simulink model "frequency_FPID_offline"  (R2025b)
settings: Solver=ode45  StartTime=0.0  StopTime=40  RelTol=1e-3
undefined symbols (not defined in the file): B1, B2, DBH1, DBH2, dbpu, GRCT1, GRCU1, KBESS, KD1, Kd1_RL, Kd2_RL, KDeng, Ke, Kev, KH1, Ki1_RL, Ki2_RL, KP, KP1, Kp1_RL, KP2, Kp2_RL, Kpc, KPV1, KPV2, Kr1, KT1, KW, Kw1, Kw2, KX1_RL, KX2_RL, KY1_RL, KY2_RL, N1, N2, Nev, PAGmax, PAGmin, R1, R2, Rev, T12, TBESS, Td0, Td1, Td2, Td3, Tev, TG1, Th1, Th2, TP1, TP2, Tpt1, Tpt2, TPV1, TPV2, Tr1, Trh1 ... (+9)
libraries: fuzblock x2, slpidlib x2, simulink x2

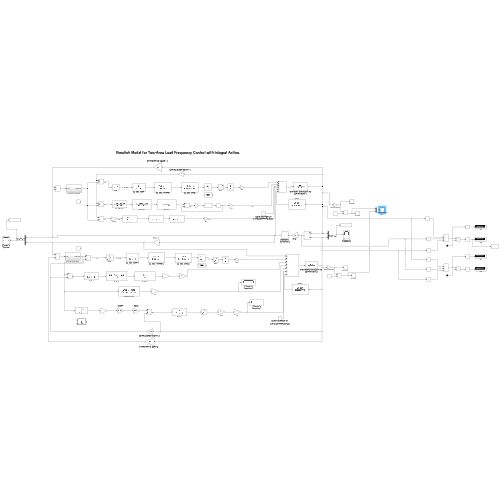
[thumbnail: Simulink's stored preview of the top-level diagram]
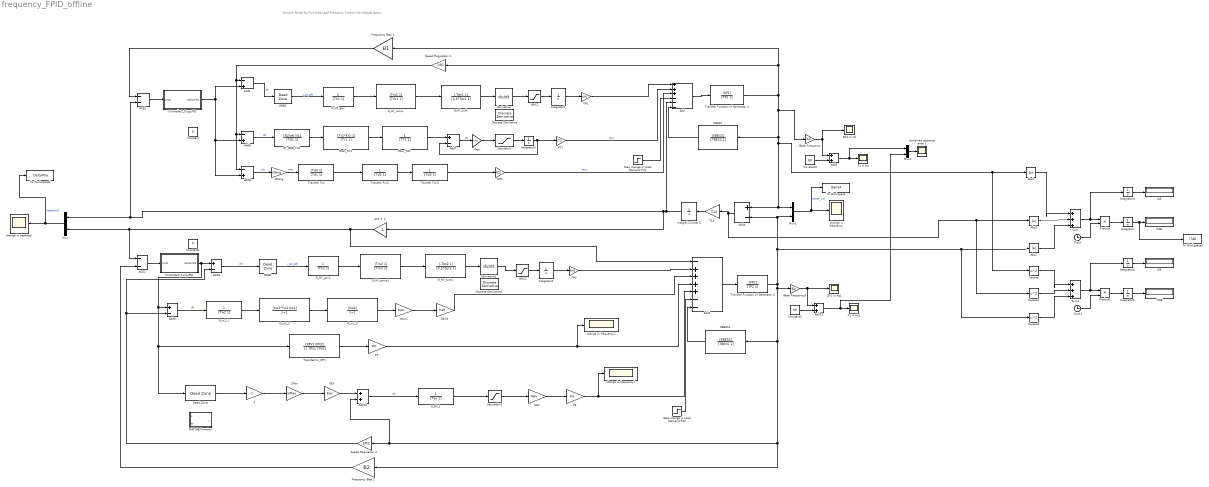
== system frequency_FPID_offline ==
  note: Simulink Model for Two-Area Load Frequency Control with Integral Action.
  " change in frequency" : Scope
      settings: ActiveDisplayYMinimum=-0.0040302316669391719  ActiveDisplayYMaximum=0.00095804845606976461
  " change in frequency1" : Scope
      settings: ActiveDisplayYMinimum=-0.00030105594584369807  ActiveDisplayYMaximum=4.6057283791285268E-5  DataLoggingVariableName=ScopeData3
  " change in frequency2" : Scope
      settings: ActiveDisplayYMinimum=-0.0033871282854349067  ActiveDisplayYMaximum=0.00055417492830862479  DataLoggingVariableName=ScopeData4
  " change in tiepower" : Scope
      settings: ActiveDisplayYMinimum=-0.0024845401904889861  ActiveDisplayYMaximum=0.0033711842064116687
  -1 : Gain  Gain=-1
  1/Rev : Gain  Gain=1/Rev
  A12 = 1 : Gain  Gain=-1
  ACE1 : Sum  Inputs=--
  ACE2 : Sum  Inputs=--
  Abs1 : Abs  SaturateOnIntegerOverflow=off
  Abs2 : Abs  SaturateOnIntegerOverflow=off
  Abs3 : Abs  SaturateOnIntegerOverflow=off
  Add : Sum  Inputs=+++---
  Add1 : Sum  Inputs=-+
  Add10 : Sum
  Add12 : Sum
  Add2 : Sum  Inputs=-++++--
  Add{3..4,7,9} (4 alike) : Sum  Inputs=+-
  Add5 : Sum
  Add6 : Sum  Inputs=-+
  Add8 : Sum  Inputs=-+
  Base Frequency : Gain  Gain=60
  Base Frequency2 : Gain  Gain=60
  Clock : Clock
  Clock1 : Clock
  Constant : Constant  Value=0
  Constant1 : Constant  Value=0
  Constant2 : Constant  Value=60
  Constant3 : Constant  Value=60
  Controller1_FuzzyPID : Subsystem
  Controller2_FuzzyPID : Subsystem
  DF1 in Hz : Scope
      settings: ActiveDisplayYMinimum=-0.70637481280735892  ActiveDisplayYMaximum=0.1303080522857864  DataLoggingVariableName=ScopeData5
  DF1 in Hz1 : Scope
      settings: ActiveDisplayYMinimum=-0.88482  ActiveDisplayYMaximum=0.09831  DataLoggingVariableName=ScopeData2
  Dead Zone : DeadZone  LowerValue=-dbpu  UpperValue=+dbpu
  Derivative : Derivative
  Derivative1 : Derivative
  Discrete Derivative : simulink/Discrete/Discrete Derivative  gainval=1.0  ICPrevScaledInput=0.0  OutMin=[]  OutMax=[]  OutDataType=fixdt(1, 16)  OutScaling=2^-10  DoSatur=off
  Discrete Derivative1 : simulink/Discrete/Discrete Derivative  gainval=1.0  ICPrevScaledInput=0.0  OutMin=[]  OutMax=[]  OutDataType=fixdt(1, 16)  OutScaling=2^-10  DoSatur=off
  F1 in Hz : Scope
      settings: ActiveDisplayYMinimum=59.317272894162173  ActiveDisplayYMaximum=60.108382672060813  DataLoggingVariableName=ScopeData7
  F1 in Hz1 : Scope
      settings: ActiveDisplayYMinimum=59.53516  ActiveDisplayYMaximum=60.11035  DataLoggingVariableName=ScopeData9
  Frequency Bias 1 : Gain  Gain=B1
  Frequency Bias 2 : Gain  Gain=B2
  GBESS : TransferFcn  Numerator=[KBESS]  Denominator=[TBESS 1]
  GBESS1 : TransferFcn  Numerator=[KBESS]  Denominator=[TBESS 1]
  GDB1 : DeadZone  LowerValue=-DBH1  UpperValue=+DBH1  ZeroCross=off
  GDB2 : DeadZone  LowerValue=-DBH2  UpperValue=+DBH2  ZeroCross=off
  GRC1 : Saturate  UpperLimit=GRCU1  LowerLimit=-GRCU1
  GRC2 : Saturate  UpperLimit=GRCU1  LowerLimit=-GRCU1
  GT_GDB_TH1 : TransferFcn  Numerator=[N2/w0 N1]  Denominator=[TG1 1]
  G_EV_1 : TransferFcn  Denominator=[Tev 1]
  G_HY_comp : TransferFcn  Numerator=[Trs1 1]  Denominator=[Trh1 1]
  G_HY_comp1 : TransferFcn  Numerator=[Trs2 1]  Denominator=[Trh2 1]
  G_HY_gov : TransferFcn  Numerator=1  Denominator=[Th1 1]
  G_HY_gov1 : TransferFcn  Numerator=1  Denominator=[Th2 1]
  G_HY_turb : TransferFcn  Numerator=[-Tpt1 1]  Denominator=[0.5*Tpt1 1]
  G_HY_turb1 : TransferFcn  Numerator=[-Tpt2 1]  Denominator=[0.5*Tpt2 1]
  G_w2_1 : TransferFcn  Denominator=[Tw2 1]
  G_w2_2 : TransferFcn  Numerator=[Kw1*Tw1 Kw1]  Denominator=[1 1]
  G_w2_3 : TransferFcn  Numerator=[Kw2]  Denominator=[1 1]
  Gain : Gain  Gain=1/Tt1
  Gain1 : Gain  Gain=Kpc
  Gain2 : Gain  Gain=KW
  Greh_TH1 : TransferFcn  Numerator=[Tr1*Kr1 1]  Denominator=[Tr1 1]
  Gtur_TH1 : TransferFcn  Denominator=[TT1 1]
  IAE : Display
  ISE : Display
  ITAE : Display
  ITSE : Display
  Integral Control 3 : Integrator
  Integrator{,1..6} (7 alike) : Integrator
  KD1 : Gain  Gain=KD1
  KDeng : Gain  Gain=KDeng
  KE : Gain  Gain=Ke
  KEV : Gain  Gain=Kev
  KH1 : Gain  Gain=KH1
  KH2 : Gain  Gain=KH1
  KP : Gain  Gain=KP
  KT1 : Gain  Gain=KT1
  MATLAB Function : MATLAB Function  TreatAsAtomicUnit=on
  Mux : Mux  Inputs=2
  Mux1 : Mux  Inputs=2
  Mux2 : Mux  Inputs=2
  NEV : Gain  Gain=Nev
  Product : Product
  Product1 : Product
  Saturation : Saturate  UpperLimit=GRCT1  LowerLimit=-GRCT1
  Saturation1 : Saturate  UpperLimit=PAGmax  LowerLimit=PAGmin
  Speed Regulation 1 : Gain  Gain=1/R1
  Speed Regulation 2 : Gain  Gain=1/R2
  Square : Math  Operator=square
  Square1 : Math  Operator=square
  Square2 : Math  Operator=square
  Step change in Load Demand Pd1 : Step  Time=0  Before=0.01  After=0.01  SampleTime=0
  Step change in Load Demand Pd2 : Step  Time=0  After=0  SampleTime=0
  Sum : Sum  Inputs=|+++
  Sum1 : Sum  Inputs=|+++
  T12 : Gain  Gain=T12
  To Workspace : ToWorkspace  VariableName=DeltaF  SaveFormat=Structure With Time
  To Workspace1 : ToWorkspace  VariableName=DeltaPtie  SaveFormat=Structure With Time  SampleTime=-1
  To Workspace2 : ToWorkspace  VariableName=ITAE  SampleTime=-1
  Transfer Fcn : TransferFcn  Numerator=[Td0 1]  Denominator=[Td1 1]
  Transfer Fcn2 : TransferFcn  Denominator=[Td2 1]
  Transfer Fcn3 : TransferFcn  Denominator=[Td3 1]
  Transfer Function of Generator 1 : TransferFcn  Numerator=[KP1]  Denominator=[TP1 1]
  Transfer Function of Generator 2 : TransferFcn  Numerator=[KP2]  Denominator=[TP2 1]
  TransferFcn_GPV : TransferFcn  Numerator=[KPV1 KPV2]  Denominator=[1 TPV1 TPV2]
  combined response area 1 : Scope
      settings: ActiveDisplayYMinimum=59.617591809890676  ActiveDisplayYMaximum=60.042588653094796  DataLoggingVariableName=ScopeData13
  wires:
  Frequency Bias 2/1 -> ACE2/2
  T12/1 -> Integral Control 3/1
  A12 = 1/1 -> Add2/1, ACE2/1, Mux/2
  Speed Regulation 2/1 -> Add9/2, Add3/2
  Mux/1 -> To Workspace1/1, " change in tiepower"/1  "DeltaPtie12"
  Add2/1 -> Transfer Function of Generator 2/1
  Mux1/1 -> To Workspace/1, " change in frequency"/1  "DeltaF_vec"
  Step change in Load Demand Pd2/1 -> Add2/6
  Speed Regulation 1/1 -> Add8/1, Add6/1, Add1/1
  Add/1 -> Transfer Function of Generator 1/1
  Step change in Load Demand Pd1/1 -> Add/4
  Frequency Bias 1/1 -> ACE1/1
  G_HY_gov/1 -> G_HY_comp/1
  Integral Control 3/1 -> ACE1/2, Mux/1, A12 = 1/1, Add/5
  Clock/1 -> Product/2
  Product/1 -> Integrator/1
  Sum/1 -> Integrator4/1, Product/1
  Integrator/1 -> To Workspace2/1, ITAE/1
  Abs1/1 -> Sum/1
  Abs3/1 -> Sum/2
  Abs2/1 -> Sum/3
  Add4/1 -> T12/1, Square1/1, Abs3/1
  GDB1/1 -> G_HY_gov/1  "u_g1_gdb"
  G_HY_turb/1 -> Derivative/1
  Derivative/1 -> GRC1/1
  GRC1/1 -> Integrator1/1
  ACE2/1 -> Controller2_FuzzyPID/1(ACE2)
  ACE1/1 -> Controller1_FuzzyPID/1(ACE1)
  Mux2/1 -> combined response area 1/1
  Constant2/1 -> Add5/2
  Base Frequency/1 -> DF1 in Hz/1, Add5/1
  Add5/1 -> Mux2/1, F1 in Hz/1
  Add12/1 -> Mux2/2, F1 in Hz1/1
  Transfer Function of Generator 2/1 -> Mux1/2, Add4/2, Square2/1, Abs2/1, Base Frequency2/1, GBESS1/1, Add10/2, Speed Regulation 2/1, Frequency Bias 2/1
  Constant3/1 -> Add12/2
  Base Frequency2/1 -> DF1 in Hz1/1, Add12/1
  G_HY_comp/1 -> G_HY_turb/1
  Integrator1/1 -> KH1/1
  KH1/1 -> Add/1
  GRC2/1 -> Integrator2/1
  G_HY_comp1/1 -> G_HY_turb1/1
  Derivative1/1 -> GRC2/1
  G_HY_gov1/1 -> G_HY_comp1/1
  G_HY_turb1/1 -> Derivative1/1
  Add3/1 -> GDB2/1  "df1"
  GDB2/1 -> G_HY_gov1/1  "u_g1_gdb"
  Integrator2/1 -> KH2/1
  KH2/1 -> Add2/2
  Add1/1 -> GDB1/1  "df1"
  Controller1_FuzzyPID/1(DeltaPref1) -> Add8/2, Add6/2, Add1/2
  Add6/1 -> GT_GDB_TH1/1  "df1"
  Greh_TH1/1 -> Gtur_TH1/1
  GT_GDB_TH1/1 -> Greh_TH1/1
  Gtur_TH1/1 -> Add7/1
  Add7/1 -> Gain/1  "df1"
  Gain/1 -> Saturation/1
  Saturation/1 -> Integrator3/1
  Integrator3/1 -> KT1/1, Add7/2
  KT1/1 -> Add/2  "Pth1"
  KDeng/1 -> Transfer Fcn/1  "Pth1"
  Transfer Fcn/1 -> Transfer Fcn2/1
  Transfer Fcn2/1 -> Transfer Fcn3/1
  Transfer Fcn3/1 -> KD1/1
  Add9/1 -> G_w2_1/1  "df1"
  G_w2_1/1 -> G_w2_2/1
  G_w2_2/1 -> G_w2_3/1
  G_w2_3/1 -> Gain1/1
  Gain1/1 -> Gain2/1
  Gain2/1 -> Add2/3
  Add8/1 -> KDeng/1  "df1"
  KD1/1 -> Add/3  "Pth1"
  TransferFcn_GPV/1 -> KP/1
  Controller2_FuzzyPID/1(DeltaPref2) -> Dead Zone/1, TransferFcn_GPV/1, Add9/1, Add3/1
  KP/1 -> " change in frequency2"/1, Add2/4
  KEV/1 -> Add10/1
  KE/1 -> " change in frequency1"/1, Add2/5
  Dead Zone/1 -> -1/1
  -1/1 -> 1/Rev/1
  1/Rev/1 -> KEV/1
  Add10/1 -> G_EV_1/1  "df1"
  G_EV_1/1 -> Saturation1/1
  Saturation1/1 -> NEV/1
  NEV/1 -> KE/1
  Transfer Function of Generator 1/1 -> Base Frequency/1, Square/1, Abs1/1, Add4/1, Mux1/1, GBESS/1, Speed Regulation 1/1, Frequency Bias 1/1
  GBESS/1 -> Add/6
  GBESS1/1 -> Add2/7
  Integrator4/1 -> IAE/1
  Integrator5/1 -> ITSE/1
  Product1/1 -> Integrator5/1
  Clock1/1 -> Product1/2
  Sum1/1 -> Integrator6/1, Product1/1
  Integrator6/1 -> ISE/1
  Square/1 -> Sum1/1
  Square1/1 -> Sum1/2
  Square2/1 -> Sum1/3

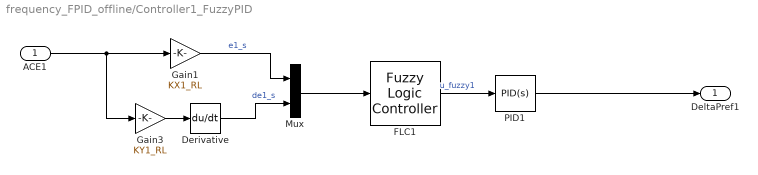
== system frequency_FPID_offline/Controller1_FuzzyPID ==
  ACE1 : Inport
  Derivative : Derivative
  FLC1 : fuzblock/Fuzzy Logic  Controller  FIS='LFC_fuzzy_trimf.fis'  OutputSampleNumber=101  DataType=double  UseLookupTable=off  NumBreakpoints=10  FuzzifiedInputs=off  RuleFiringStrengths=off  RuleOutputs=off  AggregatedOutputs=off  SimulateUsing=Interpreted execution  OutOfRangeInputValueMessage=warning  NoRuleFiredMessage=warning  EmptyOutputFuzzySetMessage=warning
  Gain1 : Gain  Gain=KX1_RL
  Gain3 : Gain  Gain=KY1_RL
  Mux : Mux  Inputs=2
  PID1 : slpidlib/PID Controller  Controller=PID  Form=Parallel  TimeDomain=Continuous-time  UseExternalTs=off  SampleTime=Ts  IntegratorMethod=Forward Euler  FilterMethod=Forward Euler  ControllerParametersSource=internal  P=Kp1_RL  I=Ki1_RL  UseKiTs=off  D=Kd1_RL  UseExternalDerivativeSource=off  N=100  UseFilter=on  TunerSelectOption=Transfer Function Based (PID Tuner App)  InitialConditionSource=internal  InitialConditionForIntegrator=0  InitialConditionForFilter=0  DifferentiatorICPrevScaledInput=0  ExternalReset=none  TrackingMode=off  Kt=1  LimitOutput=off  SatLimitsSource=internal  UpperSaturationLimit=inf  LowerSaturationLimit=-inf  LinearizeAsGain=on  AntiWindupMode=none  Kb=1  LimitIntegrator=off  UpperIntegratorSaturationLimit=inf  LowerIntegratorSaturationLimit=-inf  POutMin=[]  POutMax=[]  IOutMin=[]  IOutMax=[]  DOutMin=[]  DOutMax=[]  NOutMin=[]  NOutMax=[]  SumOutMin=[]  SumOutMax=[]  SaturationOutMin=[]  SaturationOutMax=[]  PParamMin=[]  PParamMax=[]  IParamMin=[]  IParamMax=[]  DParamMin=[]  DParamMax=[]  NParamMin=[]  NParamMax=[]  KbParamMin=[]  KbParamMax=[]  KtParamMin=[]  KtParamMax=[]  KbOutMin=[]  KbOutMax=[]  KtOutMin=[]  KtOutMax=[]  IntegratorOutMin=[]  IntegratorOutMax=[]  FilterOutMin=[]  FilterOutMax=[]  SumI1OutMin=[]  SumI1OutMax=[]  SumI2OutMin=[]  SumI2OutMax=[]  SumI3OutMin=[]  SumI3OutMax=[]  SumI4OutMin=[]  SumI4OutMax=[]  SumDOutMin=[]  SumDOutMax=[]  DifferentiatorOutMin=[]  DifferentiatorOutMax=[]  FilterDiffOutCoefMin=[]  FilterDiffOutCoefMax=[]  ReciprocalOutMin=[]  ReciprocalOutMax=[]  SumDenOutMin=[]  SumDenOutMax=[]  SumNumOutMin=[]  SumNumOutMax=[]  DivideOutMin=[]  DivideOutMax=[]  UdiffTsProdOutMin=[]  UdiffTsProdOutMax=[]  NTsProdOutMin=[]  NTsProdOutMax=[]  UintegralTsProdOutMin=[]  UintegralTsProdOutMax=[]  UngainTsProdOutMin=[]  UngainTsProdOutMax=[]  ClampingZeroOutDataTypeStr=Inherit: Inherit via back propagation  ClampingZeroOutMin=[]  ClampingZeroOutMax=[]  FilterDenConstantOutDataTypeStr=Inherit: Inherit via back propagation  FilterDenConstantOutMin=[]  FilterDenConstantOutMax=[]  PCopyOutDataTypeStr=Inherit: Inherit via back propagation  PCopyOutMin=[]  PCopyOutMax=[]  NCopyOutDataTypeStr=Inherit: Inherit via back propagation  NCopyOutMin=[]  NCopyOutMax=[]  IntegratorContinuousStateAttributes=''  IntegratorStateMustResolveToSignalObject=off  IntegratorRTWStateStorageClass=Auto  FilterContinuousStateAttributes=''  FilterStateMustResolveToSignalObject=off  FilterRTWStateStorageClass=Auto  ParallelPVariant=InternalParameters  IdealPVariant=Disabled  IVariant=InternalParameters  DVariant=InternalParameters  IntegratorVariant=Continuous  SatVariant=Disabled  AWVariant=Passthrough  PCopyVariant=Disabled  TRVariant=Disabled  FdbkBlocksVariant=Forward  IdealPFdbkVariant=Disabled  SatFdbkVariant=Disabled  DerivativeFilterVariant=ContFilter  NVariant=InternalParameters  NCopyVariant=Disabled  FilterICVariant=InternalICsFilter  IntegratorICVariant=InternalICs  ExternalResetVariant=Disabled  TRSumVariant=Passthrough  SumFdbkVariant=Disabled  SumVariant=Sum_PID  TsampFilterVariant=InternalTs  TsampNgainVariant=Passthrough  TsampIntegralVariant=Disabled_SignalSpec  ExternalSaturationOutDataTypeStr=Inherit: Same as second input  DerivativeSourceVariant=ErrorSignal  PreIntVariant=InternalPreInt
  DeltaPref1 : Outport
  wires:
  PID1/1 -> DeltaPref1/1
  ACE1/1 -> Gain1/1, Gain3/1
  Gain1/1 -> Mux/1  "e1_s"
  Derivative/1 -> Mux/2  "de1_s"
  Mux/1 -> FLC1/1
  FLC1/1 -> PID1/1  "u_fuzzy1"
  Gain3/1 -> Derivative/1

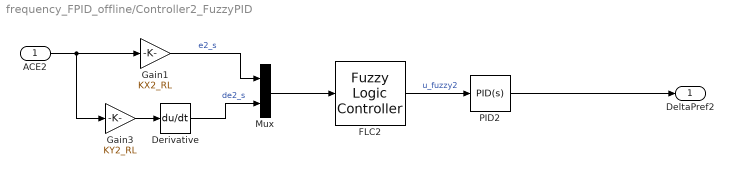
== system frequency_FPID_offline/Controller2_FuzzyPID ==
  ACE2 : Inport
  Derivative : Derivative
  FLC2 : fuzblock/Fuzzy Logic  Controller  FIS='LFC_fuzzy_trimf.fis'  OutputSampleNumber=101  DataType=double  UseLookupTable=off  NumBreakpoints=10  FuzzifiedInputs=off  RuleFiringStrengths=off  RuleOutputs=off  AggregatedOutputs=off  SimulateUsing=Interpreted execution  OutOfRangeInputValueMessage=warning  NoRuleFiredMessage=warning  EmptyOutputFuzzySetMessage=warning
  Gain1 : Gain  Gain=KX2_RL
  Gain3 : Gain  Gain=KY2_RL
  Mux : Mux  Inputs=2
  PID2 : slpidlib/PID Controller  Controller=PID  Form=Parallel  TimeDomain=Continuous-time  UseExternalTs=off  SampleTime=Ts  IntegratorMethod=Forward Euler  FilterMethod=Forward Euler  ControllerParametersSource=internal  P=Kp2_RL  I=Ki2_RL  UseKiTs=off  D=Kd2_RL  UseExternalDerivativeSource=off  N=100  UseFilter=on  TunerSelectOption=Transfer Function Based (PID Tuner App)  InitialConditionSource=internal  InitialConditionForIntegrator=0  InitialConditionForFilter=0  DifferentiatorICPrevScaledInput=0  ExternalReset=none  TrackingMode=off  Kt=1  LimitOutput=off  SatLimitsSource=internal  UpperSaturationLimit=inf  LowerSaturationLimit=-inf  LinearizeAsGain=on  AntiWindupMode=none  Kb=1  LimitIntegrator=off  UpperIntegratorSaturationLimit=inf  LowerIntegratorSaturationLimit=-inf  POutMin=[]  POutMax=[]  IOutMin=[]  IOutMax=[]  DOutMin=[]  DOutMax=[]  NOutMin=[]  NOutMax=[]  SumOutMin=[]  SumOutMax=[]  SaturationOutMin=[]  SaturationOutMax=[]  PParamMin=[]  PParamMax=[]  IParamMin=[]  IParamMax=[]  DParamMin=[]  DParamMax=[]  NParamMin=[]  NParamMax=[]  KbParamMin=[]  KbParamMax=[]  KtParamMin=[]  KtParamMax=[]  KbOutMin=[]  KbOutMax=[]  KtOutMin=[]  KtOutMax=[]  IntegratorOutMin=[]  IntegratorOutMax=[]  FilterOutMin=[]  FilterOutMax=[]  SumI1OutMin=[]  SumI1OutMax=[]  SumI2OutMin=[]  SumI2OutMax=[]  SumI3OutMin=[]  SumI3OutMax=[]  SumI4OutMin=[]  SumI4OutMax=[]  SumDOutMin=[]  SumDOutMax=[]  DifferentiatorOutMin=[]  DifferentiatorOutMax=[]  FilterDiffOutCoefMin=[]  FilterDiffOutCoefMax=[]  ReciprocalOutMin=[]  ReciprocalOutMax=[]  SumDenOutMin=[]  SumDenOutMax=[]  SumNumOutMin=[]  SumNumOutMax=[]  DivideOutMin=[]  DivideOutMax=[]  UdiffTsProdOutMin=[]  UdiffTsProdOutMax=[]  NTsProdOutMin=[]  NTsProdOutMax=[]  UintegralTsProdOutMin=[]  UintegralTsProdOutMax=[]  UngainTsProdOutMin=[]  UngainTsProdOutMax=[]  ClampingZeroOutDataTypeStr=Inherit: Inherit via back propagation  ClampingZeroOutMin=[]  ClampingZeroOutMax=[]  FilterDenConstantOutDataTypeStr=Inherit: Inherit via back propagation  FilterDenConstantOutMin=[]  FilterDenConstantOutMax=[]  PCopyOutDataTypeStr=Inherit: Inherit via back propagation  PCopyOutMin=[]  PCopyOutMax=[]  NCopyOutDataTypeStr=Inherit: Inherit via back propagation  NCopyOutMin=[]  NCopyOutMax=[]  IntegratorContinuousStateAttributes=''  IntegratorStateMustResolveToSignalObject=off  IntegratorRTWStateStorageClass=Auto  FilterContinuousStateAttributes=''  FilterStateMustResolveToSignalObject=off  FilterRTWStateStorageClass=Auto  ParallelPVariant=InternalParameters  IdealPVariant=Disabled  IVariant=InternalParameters  DVariant=InternalParameters  IntegratorVariant=Continuous  SatVariant=Disabled  AWVariant=Passthrough  PCopyVariant=Disabled  TRVariant=Disabled  FdbkBlocksVariant=Forward  IdealPFdbkVariant=Disabled  SatFdbkVariant=Disabled  DerivativeFilterVariant=ContFilter  NVariant=InternalParameters  NCopyVariant=Disabled  FilterICVariant=InternalICsFilter  IntegratorICVariant=InternalICs  ExternalResetVariant=Disabled  TRSumVariant=Passthrough  SumFdbkVariant=Disabled  SumVariant=Sum_PID  TsampFilterVariant=InternalTs  TsampNgainVariant=Passthrough  TsampIntegralVariant=Disabled_SignalSpec  ExternalSaturationOutDataTypeStr=Inherit: Same as second input  DerivativeSourceVariant=ErrorSignal  PreIntVariant=InternalPreInt
  DeltaPref2 : Outport
  wires:
  PID2/1 -> DeltaPref2/1
  Gain3/1 -> Derivative/1
  Mux/1 -> FLC2/1
  ACE2/1 -> Gain1/1, Gain3/1
  Derivative/1 -> Mux/2  "de2_s"
  FLC2/1 -> PID2/1  "u_fuzzy2"
  Gain1/1 -> Mux/1  "e2_s"

== matlab function frequency_FPID_offline/MATLAB Function ==
  data: u input; y output; db input
function y = dband(u, db)
% u: Hz, db: Hz
if abs(u) < db
    y = 0;
else
    y = u;   % giữ nguyên biên độ ngoài deadband
end
end
